simulink model "lfp_cell_2rc"  (R2025a)
settings: Solver=FixedStepDiscrete  StartTime=0.0  StopTime=3600  FixedStep=dt  RelTol=1e-3
InitFcn:
  | if ~exist('p','var'), p = lfp.cellParams(); end
  | if ~exist('dt','var'), dt = 1; end
  | if ~exist('T_amb','var'), T_amb = 25; end
  | if ~exist('iProfile','var'), iProfile = [0 6; 3600 6]; end
undefined symbols (not defined in the file): dt, p, T_amb
settings Model: Creator=hari2  LastModifiedBy=hari2
settings DataIOCC: SaveOutput=off  SaveTime=off

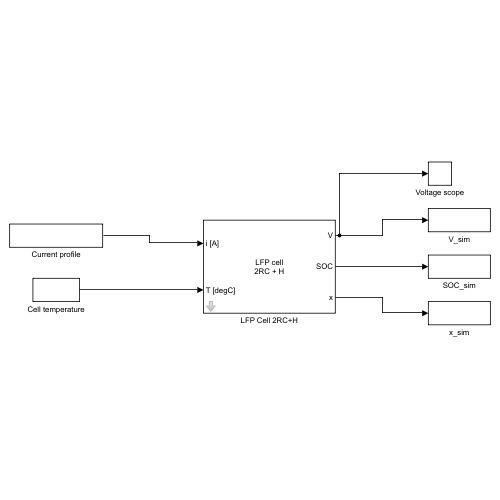
[thumbnail: Simulink's stored preview of the top-level diagram]
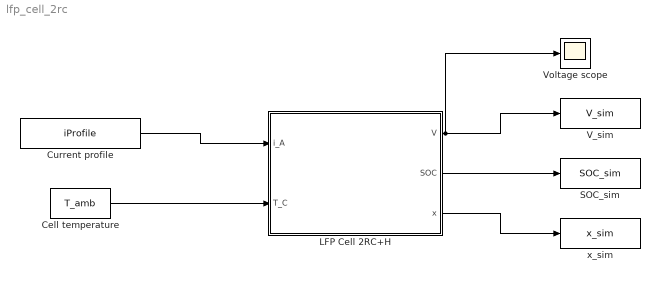
== system lfp_cell_2rc ==
  Cell temperature : Constant  Value=T_amb
  Current profile : FromWorkspace  VariableName=iProfile  SampleTime=dt  Interpolate=off  OutputAfterFinalValue=Holding final value
  LFP Cell 2RC+H : Subsystem  mask(LFP cell (2RC + hysteresis)){SOC0=1}
      mask prompts: SOC0 "Initial SOC [0-1]"
      mask help: Discrete 2RC equivalent-circuit LFP cell with one-state hysteresis. Parameters: workspace struct p = lfp.cellParams(), step dt [s]. Inputs: current [A] (+ = discharge), temperature [degC].
      mask Display:
      | disp('LFP cell\n2RC + H');
      | port_label('input',1,'i [A]');
      | port_label('input',2,'T [degC]');
      | port_label('output',1,'V');
      | port_label('output',2,'SOC');
      | port_label('output',3,'x');
  SOC_sim : ToWorkspace  VariableName=SOC_sim  SampleTime=-1
  V_sim : ToWorkspace  VariableName=V_sim  SampleTime=-1
  Voltage scope : Scope
  x_sim : ToWorkspace  VariableName=x_sim  SampleTime=-1
  wires:
  Current profile/1 -> LFP Cell 2RC+H/1(i_A)
  Cell temperature/1 -> LFP Cell 2RC+H/2(T_C)
  LFP Cell 2RC+H/1(V) -> V_sim/1, Voltage scope/1
  LFP Cell 2RC+H/2(SOC) -> SOC_sim/1
  LFP Cell 2RC+H/3(x) -> x_sim/1

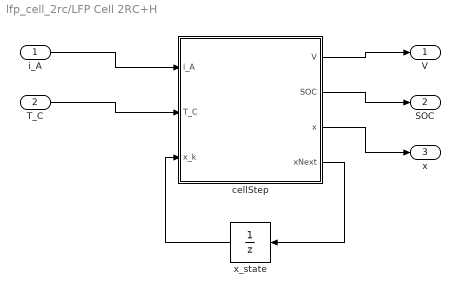
== system lfp_cell_2rc/LFP Cell 2RC+H ==
  i_A : Inport
  T_C : Inport  Port=2
  cellStep : MATLAB Function  TreatAsAtomicUnit=on
  x_state : UnitDelay  InitialCondition=[SOC0; 0; 0; 0]  SampleTime=dt  HasFrameUpgradeWarning=on
  V : Outport
  SOC : Outport  Port=2
  x : Outport  Port=3
  wires:
  i_A/1 -> cellStep/1(i_A)
  T_C/1 -> cellStep/2(T_C)
  x_state/1 -> cellStep/3(x_k)
  cellStep/4(xNext) -> x_state/1
  cellStep/1(V) -> V/1
  cellStep/2(SOC) -> SOC/1
  cellStep/3(x) -> x/1

== matlab function lfp_cell_2rc/LFP Cell 2RC+H/cellStep ==
  data: i_A input double size=1; V output double size=1; T_C input double size=1; x_k input double size=[4 1]; SOC output double size=1; x output double size=[4 1]; xNext output double size=[4 1]; p parameter; dt parameter
function [V, SOC, x, xNext] = cellStep(i_A, T_C, x_k, p, dt)
%#codegen
% One step of the LFP 2RC + hysteresis model (same code as the MATLAB scripts).
%   i_A : cell current [A], + = discharge     T_C : cell temperature [degC]
%   x_k : state [soc; v1; v2; h] from the Unit Delay
[xNext, V] = lfp.cellStep(x_k, i_A, T_C, dt, p);
SOC = x_k(1);
x   = x_k;
